simulink model "commande_IGBT"  (Simulink 7.4)
settings: Solver=FixedStepDiscrete  StartTime=0.0  StopTime=inf  FixedStep=1/1200  RelTol=1e-3
undefined symbols (not defined in the file or in its folder): ANmax, OC1max, OC2max, OC3max
libraries: dsPICdrivers x5
settings Model: Creator=Lubin  LastModifiedBy=ELMAY
settings OptimizationCC: InitFltsAndDblsToZero=on  OptimizeModelRefInitCode=on  LifeSpan=1
settings DebuggingCC: SaveWithParameterizedLinksMsg=none  SignalResolutionControl=TryResolveAllWithWarning  InheritedTsInSrcMsg=none  IntegerOverflowMsg=none  ParameterOverflowMsg=none
settings HardwareCC: ProdBitPerInt=16  ProdEndianess=LittleEndian  ProdWordSize=16  ProdHWDeviceType=16-bit Generic  TargetHWDeviceType=32-bit Generic
settings RTWCC: SystemTargetFile=dspic.tlc  MakeCommand=make_CreateMPLAB  TemplateMakefile=dspic_pic30_gcc.tmf  PostCodeGenCommand=dsPIC_Compile()  Description=Embedded Target for Microchip dsPIC (real-time)  ProcessScript=dspic_make_rtw_hook
settings CodeAppCC: IgnoreCustomStorageClasses=off
settings STFCustomTargetCC: IncludeMdlTerminateFcn=off  CombineOutputUpdateFcns=on  SuppressErrorStatus=on  ERTCustomFileBanners=on  SupportContinuousTime=off  SupportNonInlinedSFcns=off  SystemTargetFile=dspic.tlc
settings ERTTargetCC: MultiwordLength=2048  ParMdlRefBuildCompliant=off  CompOptLevelCompliant=off  IncludeMdlTerminateFcn=off  SuppressErrorStatus=on  ERTFirstTimeCompliant=off  ModelStepFunctionPrototypeControlCompliant=off  CPPClassGenCompliant=off  InlinedParameterPlacement=NonHierarchical  ERTSrcFileBannerTemplate=dsPIC_code_template.cgt  ERTHdrFileBannerTemplate=dsPIC_code_template.cgt  ERTDataSrcFileTemplate=dsPIC_code_template.cgt  ERTDataHdrFileTemplate=dsPIC_code_template.cgt  ERTCustomFileTemplate=dsPIC_main.tlc  ConvertIfToSwitch=off
settings CustomProperty: DataType=string  Value=D:\PROGRA~1\MATLAB\R2009b\bin\win32\gmake

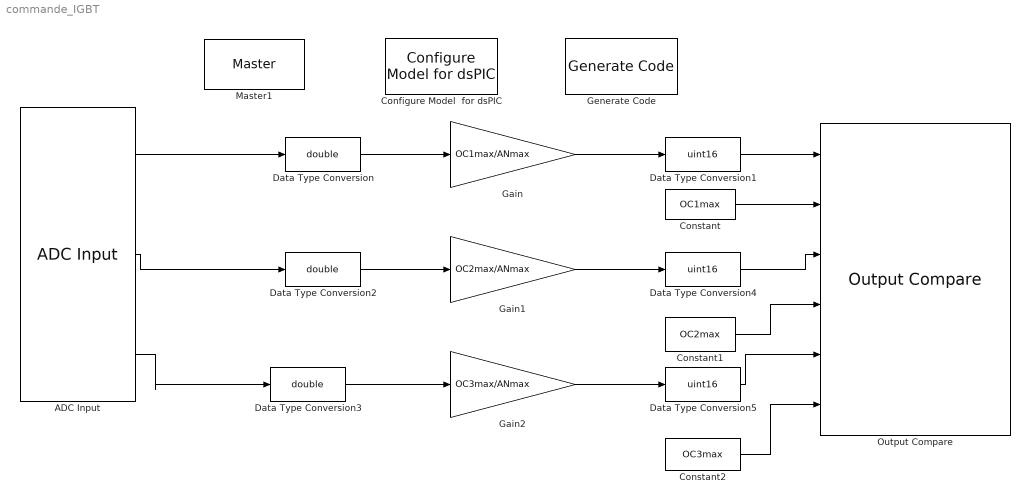
== system commande_IGBT ==
  ADC Input : dsPICdrivers/Peripheral I//O/ADC Input  Tag=dsPIC_ADC  Priority=5  ADC_TYPE=12 bits  ADC_MODE=Continuous sampling & get last channel value  NbrSampleStep=1  VoltRefpopup="AVdd  -  AVss"  OutFormatBitspopup=0000 dddd dddd dddd : Integer  InterruptPriority=6  ANCHANNELS=[0 1 2]  MaxName=ANmax = 4095  Rin=5e2  ADCS=1  SAMC=1  Temperature=25  DMAChannel=0  SampleTime=-1  Status="OK  |  Tsmp=1.000e-006 |  T/Channel=1.500e-005 |  Tall=4.500e-005"  SSRC=auto convert
  Configure Model  for dsPIC : dsPICdrivers/Simulink Configuration/Configure Model  for dsPIC
  Constant : Constant  Value=OC1max  OutDataTypeMode=uint16  OutDataType=sfix(16)  OutScaling=2^0  OutDataTypeStr=uint16
  Constant1 : Constant  Value=OC2max  OutDataTypeMode=uint16  OutDataType=sfix(16)  OutScaling=2^0  OutDataTypeStr=uint16
  Constant2 : Constant  Value=OC3max  OutDataTypeMode=uint16  OutDataType=sfix(16)  OutScaling=2^0  OutDataTypeStr=uint16
  Data Type Conversion : DataTypeConversion  OutDataTypeMode=double  OutDataType=sfix(16)  OutScaling=2^0  OutDataTypeStr=double
  Data Type Conversion1 : DataTypeConversion  OutDataTypeMode=uint16  OutDataType=sfix(16)  OutScaling=2^0  OutDataTypeStr=uint16
  Data Type Conversion2 : DataTypeConversion  OutDataTypeMode=double  OutDataType=sfix(16)  OutScaling=2^0  OutDataTypeStr=double
  Data Type Conversion3 : DataTypeConversion  OutDataTypeMode=double  OutDataType=sfix(16)  OutScaling=2^0  OutDataTypeStr=double
  Data Type Conversion4 : DataTypeConversion  OutDataTypeMode=uint16  OutDataType=sfix(16)  OutScaling=2^0  OutDataTypeStr=uint16
  Data Type Conversion5 : DataTypeConversion  OutDataTypeMode=uint16  OutDataType=sfix(16)  OutScaling=2^0  OutDataTypeStr=uint16
  Gain : Gain  Gain=OC1max/ANmax  ParameterDataTypeMode=double  ParameterDataType=sfix(16)  ParameterScaling=2^0  ParamDataTypeStr=double  OutDataType=sfix(16)  OutScaling=2^0
  Gain1 : Gain  Gain=OC2max/ANmax  ParameterDataTypeMode=double  ParameterDataType=sfix(16)  ParameterScaling=2^0  ParamDataTypeStr=double  OutDataType=sfix(16)  OutScaling=2^0
  Gain2 : Gain  Gain=OC3max/ANmax  ParameterDataTypeMode=double  ParameterDataType=sfix(16)  ParameterScaling=2^0  ParamDataTypeStr=double  OutDataType=sfix(16)  OutScaling=2^0
  Generate Code : dsPICdrivers/Simulink Configuration/Generate Code
  Master1 : dsPICdrivers/Master  Tag=dsPIC_MASTER  Priority=1  TimeStepType=Timer1  picType=30f4013  fcy=1e6  Quartz_33f=5e6  PLLActive_33f=off  fcyDesired_33f=0  tmr1="[1  832  0.04]"  tmr1Info="Time Step : 0.000833  ;   Error : 0.04%  PR1=832"  tmr2345="[1  0  0  0]"  tmr2345cfg=[-1 -1 -1 -1]  IOautoConf=on  typePort="[ 0  0  0  0  0  0  0  0  0  0  0  0  0  0  0  0  8  8  8  0  0  0  0  0  0  0  0  0  0  0  0  0  0  0  0  0  0  0  0  0  0  0  0  0  0  0  0  0  7  7  7  0  0  0  0  0  0  0  0  0  0  0  0  0  0  0  0  0  0  0  0  0  0  0  0  0  0  0  0  0  0  0  0  0  0  0  0  0  0  0  0  0  0  0  0  0  0  0  0  0  0  0  0  0  0  0  0  0  0  0  0  0 ]"  TRIS="[ 65535  65535  65535  65528  65535  65535  65535 ]"  ADPCFG=0  MasterBusyPort=None  MasterOverloadPort=None  FOSC=HS  ClockSwitchMonitor=Both disabled  TempProtection_33f=TEMP_ON  FPBOR=PBOR_OFF  PWRT=PWRT_OFF  MCLR=MCLR_DIS  ICD=ICS_PGD1  JTAGEN=JTAGEN_OFF  PowerSave=off  OverrideFcy=off  NewFcy=1e6  PR2345="[65535  65535  65535  65535]"
  Output Compare : dsPICdrivers/Peripheral I//O/Output Compare  Tag=dsPIC_PWM_out  Priority=5  IntPriority=3  CHANNEL=[1 2 3]  Channel_UP_Down_Periode="[5  5  5]"  MaxChannel="[0.02        0.02        0.02]"  MaxName=' OC1max , OC2max , OC3max '  Precision="[14.2876      14.2876      14.2876]"  Timer="[2  2  2]"  Status=OK  SafeMarge="[0  0  0]"  PortLetter="[68  68  68]"  PortNumber="[0  1  2]"  MaxValues="[19999  19999  19999]"
  wires:
  ADC Input/1 -> Data Type Conversion/1
  Gain/1 -> Data Type Conversion1/1
  Data Type Conversion/1 -> Gain/1
  Constant/1 -> Output Compare/2
  Data Type Conversion1/1 -> Output Compare/1
  ADC Input/2 -> Data Type Conversion2/1
  ADC Input/3 -> Data Type Conversion3/1
  Data Type Conversion2/1 -> Gain1/1
  Gain1/1 -> Data Type Conversion4/1
  Data Type Conversion4/1 -> Output Compare/3
  Data Type Conversion3/1 -> Gain2/1
  Gain2/1 -> Data Type Conversion5/1
  Data Type Conversion5/1 -> Output Compare/5
  Constant1/1 -> Output Compare/4
  Constant2/1 -> Output Compare/6
